simulink model "LQ_6DOF_V3"  (R2025b)
settings: Solver=VariableStepAuto  StartTime=0.0  StopTime=27.7  RelTol=1e-3
undefined symbols (not defined in the file): AVI, bp, cg, dcg_dMfu_table, dcg_dMox_table, dI_dMfu_table, dI_dMox_table, ENGINE, fu_masses, IN, K1flat, K2grid, MoI, OUT, ox_masses, TANKS, Target_Trajectory, tbl1, tbl2, tgrid, unom
libraries: aerolibanim x1, dspindex x1, matrix_library x1
settings Model: Creator=maxma  LastModifiedBy=maxma

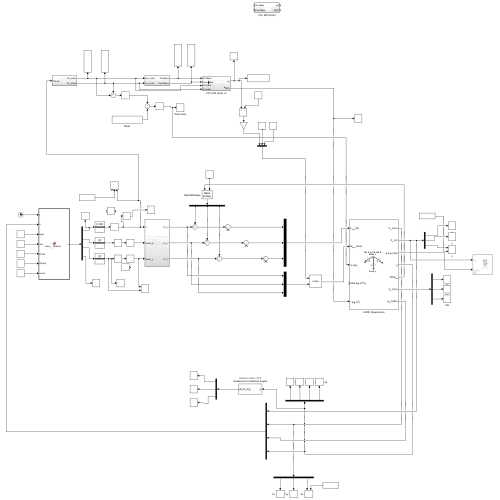
[thumbnail: Simulink's stored preview of the top-level diagram]
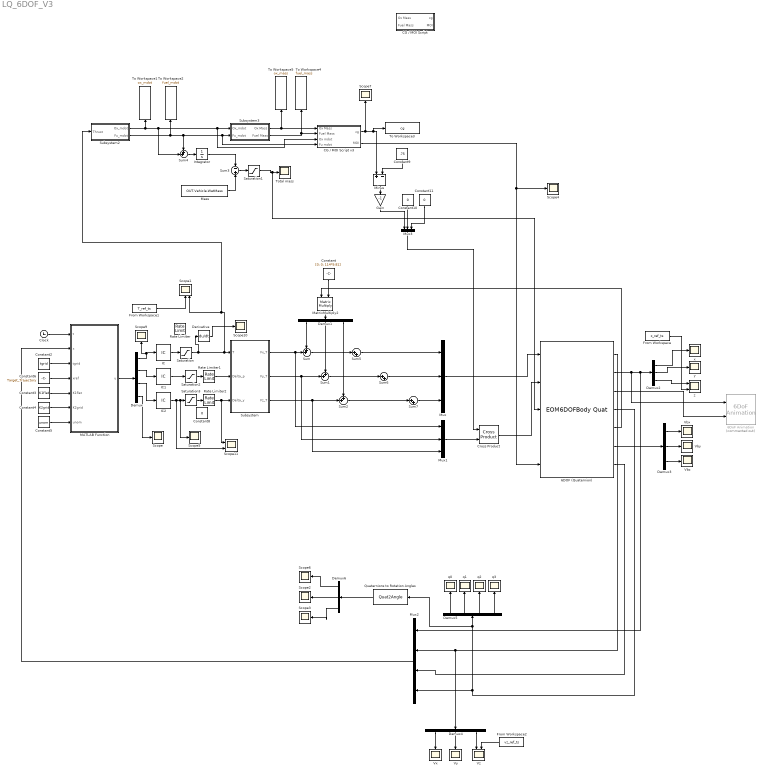
== system LQ_6DOF_V3 ==
  6DOF (Quaternion) : EOM6DOFBodyQuat  mtype=Custom Variable  eul_0=[pi/16 pi/2 pi/16]  mass_0=114  inertia=[16.5 0 0; 0 16.5 0; 0 0 16.5]
  6DoF Animation : aerolibanim/6DoF Animation  Commented=on  u1=[0 200 -200 200 -100 5]  u2=0.1  u3=2  u4=[4000 0 -5000]  u5=Fly alongside  u6=[100 100 -50]  u7=10  u8=on
  CG / MOI Script : Subsystem
  CG / MOI Script v3 : Subsystem
  Clock : Clock
  Constant : Constant  Value=[0; 0; 114*9.81]
  Constant10 : Constant  Value=0
  Constant11 : Constant  Value=0
  Constant2 : Constant  Value=tgrid
  Constant3 : Constant  Value=K1flat
  Constant4 : Constant  Value=K2grid
  Constant5 : Constant  Value=unom
  Constant6 : Constant  Value=Target_Trajectory
  Constant8 : Constant  Value=0
  Constant9 : Constant  Value=.75
  Cross Product : matrix_library/Cross Product
  Demux : Demux
  Demux{1..4,6} (5 alike) : Demux  Outputs=3
  Demux5 : Demux
  Derivative : Derivative  CoefficientInTFapproximation=10^-3
  From Workspace : FromWorkspace  VariableName=z_ref_ts
  From Workspace1 : FromWorkspace  VariableName=T_ref_ts
  From Workspace2 : FromWorkspace  VariableName=vz_ref_ts
  Gain : Gain  Gain=-1
  IC : InitialCondition  Value=1300
  IC1 : InitialCondition  Value=0
  IC2 : InitialCondition  Value=0
  Integrator : Integrator
  MATLAB Function : MATLAB Function  TreatAsAtomicUnit=on
  Mass : Constant  Value=OUT.Vehicle.WetMass
  MatrixMultiply2 : Product  Multiplication=Matrix(*)
  Minus : Sum  Inputs=+-
  Mux : Mux  Inputs=3
  Mux1 : Mux  Inputs=3
  Mux2 : Mux
  Mux3 : Mux  Inputs=3
  Quaternions to Rotation Angles : Quat2Angle
      settings: AttributesFormatString=Rotation Order: %<rotationOrder>
  Rate Limiter : RateLimiter  RisingSlewLimit=400  FallingSlewLimit=-400  SampleTimeMode=inherited
  Rate Limiter1 : RateLimiter  RisingSlewLimit=30*(pi/180)  FallingSlewLimit=-30*(pi/180)  SampleTimeMode=inherited
  Rate Limiter2 : RateLimiter  RisingSlewLimit=30*(pi/180)  FallingSlewLimit=-30*(pi/180)  SampleTimeMode=inherited
  Saturation : Saturate  UpperLimit=2400  LowerLimit=890
  Saturation1 : Saturate  UpperLimit=OUT.Vehicle.WetMass  LowerLimit=OUT.Vehicle.DryMass
  Saturation2 : Saturate  UpperLimit=7.5*(pi/180)  LowerLimit=-7.5*(pi/180)
  Saturation3 : Saturate  UpperLimit=7.5*(pi/180)  LowerLimit=-7.5*(pi/180)
  Scope{,2..7,9..10} (9 alike) : Scope
      Scope settings: ActiveDisplayYMinimum=-3.0324843779906377E-12  ActiveDisplayYMaximum=5.2601576594002828E-13  DataLoggingVariableName=ScopeData16
      Scope10 settings: ActiveDisplayYMinimum=-65.775875066860962  ActiveDisplayYMaximum=70.502667630153027  DataLoggingVariableName=ScopeData25
      Scope2 settings: ActiveDisplayYMinimum=1.5707657022295076  ActiveDisplayYMaximum=1.5707997295243843  DataLoggingVariableName=ScopeData17
      Scope3 settings: ActiveDisplayYMinimum=-3.9269859448764697  ActiveDisplayYMaximum=3.926989958417944  DataLoggingVariableName=ScopeData18
      Scope4 settings: ActiveDisplayYMinimum=-4.8001439667860453  ActiveDisplayYMaximum=43.201295701074415  DataLoggingVariableName=ScopeData4
      Scope5 settings: ActiveDisplayYMinimum=-1  ActiveDisplayYMaximum=1  DataLoggingVariableName=ScopeData5
      Scope6 settings: ActiveDisplayYMinimum=-3.9269859448764652  ActiveDisplayYMaximum=3.9269899584179448  DataLoggingVariableName=ScopeData19
      Scope7 settings: ActiveDisplayYMinimum=0.92832100501550818  ActiveDisplayYMaximum=1.0480775142034395  DataLoggingVariableName=ScopeData20
      Scope9 settings: DataLoggingVariableName=ScopeData24
  Scope1 : Scope  NumInputPorts=3
      settings: ActiveDisplayYMinimum=-771.02753736758768  ActiveDisplayYMaximum=3013.6766717670284
  Scope11 : Scope  NumInputPorts=2
      settings: ActiveDisplayYMinimum=-2.8831472481064673E-8  ActiveDisplayYMaximum=2.8689575203909038E-8  DataLoggingVariableName=ScopeData26
  Subsystem : Subsystem
  Subsystem2 : Subsystem
  Subsystem3 : Subsystem
  Sum{,1..2,4} (4 alike) : Sum  Inputs=++|
  Sum3 : Sum  Inputs=-|+
  Sum5 : Sum  Inputs=|++
  Sum6 : Sum  Inputs=|++
  Sum7 : Sum  Inputs=|++
  To Workspace1 : ToWorkspace  VariableName=ox_mdot  SaveFormat=Timeseries  SampleTime=-1
  To Workspace2 : ToWorkspace  VariableName=fuel_mdot  SaveFormat=Timeseries  SampleTime=-1
  To Workspace3 : ToWorkspace  VariableName=cg  SaveFormat=Timeseries  SampleTime=-1
  To Workspace4 : ToWorkspace  VariableName=fuel_mass  SaveFormat=Timeseries  SampleTime=-1
  To Workspace5 : ToWorkspace  VariableName=ox_mass  SaveFormat=Timeseries  SampleTime=-1
  Total mass : Scope
      settings: ActiveDisplayYMinimum=13.754311330723397  ActiveDisplayYMaximum=213.7543113307234  DataLoggingVariableName=ScopeData23
  Vbx : Scope
      settings: ActiveDisplayYMinimum=-1  ActiveDisplayYMaximum=1  DataLoggingVariableName=ScopeData6
  Vby : Scope
      settings: ActiveDisplayYMinimum=-1  ActiveDisplayYMaximum=1  DataLoggingVariableName=ScopeData7
  Vbz : Scope
      settings: ActiveDisplayYMinimum=-1  ActiveDisplayYMaximum=1  DataLoggingVariableName=ScopeData8
  Vx : Scope
      settings: ActiveDisplayYMinimum=-1  ActiveDisplayYMaximum=1  DataLoggingVariableName=ScopeData9
  Vy : Scope
      settings: DataLoggingVariableName=ScopeData10
  Vz : Scope  NumInputPorts=2
      settings: ActiveDisplayYMinimum=-7.8986716750089583  ActiveDisplayYMaximum=3.7459269640586941  DataLoggingVariableName=ScopeData11
  q{0..3} (4 alike) : Scope
      q0 settings: ActiveDisplayYMinimum=-1  ActiveDisplayYMaximum=1  DataLoggingVariableName=ScopeData12
      q1 settings: ActiveDisplayYMinimum=-1  ActiveDisplayYMaximum=1  DataLoggingVariableName=ScopeData13
      q2 settings: ActiveDisplayYMinimum=-1  ActiveDisplayYMaximum=1  DataLoggingVariableName=ScopeData14
      q3 settings: ActiveDisplayYMinimum=-1  ActiveDisplayYMaximum=1  DataLoggingVariableName=ScopeData15
  x : Scope
      settings: ActiveDisplayYMinimum=-1  ActiveDisplayYMaximum=1
  y : Scope
      settings: ActiveDisplayYMinimum=-1  ActiveDisplayYMaximum=1  DataLoggingVariableName=ScopeData2
  z : Scope  NumInputPorts=2
      settings: ActiveDisplayYMinimum=-33.672522393176216  ActiveDisplayYMaximum=3.7425921324673848  DataLoggingVariableName=ScopeData3
  wires:
  6DOF (Quaternion)/2 -> 6DoF Animation/1, Demux2/1, Mux2/1
  Subsystem/1(Fx_T) -> Sum/2, Mux1/1
  Subsystem/2(Fy_T) -> Sum1/2, Mux1/2
  Subsystem/3(Fz_T) -> Sum2/2, Mux1/3
  Mux/1 -> 6DOF (Quaternion)/1
  MatrixMultiply2/1 -> Demux1/1
  Cross Product/1 -> 6DOF (Quaternion)/2
  6DOF (Quaternion)/5 -> MatrixMultiply2/1
  6DOF (Quaternion)/6 -> Demux3/1
  6DOF (Quaternion)/7 -> Mux2/3
  6DOF (Quaternion)/1 -> Demux4/1, Mux2/2
  6DOF (Quaternion)/4 -> Mux2/4, Quaternions to Rotation Angles/1, Demux5/1
  MATLAB Function/1(u) -> Demux/1
  Demux/1 -> Scope9/1, IC/1
  Demux/2 -> IC1/1
  Demux/3 -> IC2/1
  Mux2/1 -> MATLAB Function/2(x)
  Constant2/1 -> MATLAB Function/3(tgrid)
  Clock/1 -> MATLAB Function/1(t)
  Constant6/1 -> MATLAB Function/4(xref)
  Constant3/1 -> MATLAB Function/5(K1flat)
  Constant4/1 -> MATLAB Function/6(K2grid)
  Constant5/1 -> MATLAB Function/7(unom)
  Constant/1 -> MatrixMultiply2/2
  IC2/1 -> Scope11/2, Scope5/1, Saturation3/1
  IC1/1 -> Saturation2/1
  IC/1 -> Saturation/1
  Demux1/1 -> Sum/1
  Demux1/2 -> Sum1/1
  Demux1/3 -> Sum2/1
  6DOF (Quaternion)/3 -> 6DoF Animation/2
  Demux2/1 -> x/1
  Demux2/2 -> y/1
  Demux2/3 -> z/1
  Demux3/3 -> Vbz/1
  Demux3/2 -> Vby/1
  Demux3/1 -> Vbx/1
  Demux4/1 -> Vx/1
  Demux4/2 -> Vy/1
  Demux4/3 -> Vz/1
  Demux5/2 -> q1/1
  Demux5/4 -> q3/1
  Demux5/3 -> q2/1
  Demux5/1 -> q0/1
  From Workspace/1 -> z/2
  From Workspace1/1 -> Scope1/2
  Demux/4 -> Scope/1
  Mux1/1 -> Cross Product/2
  From Workspace2/1 -> Vz/2
  Quaternions to Rotation Angles/1 -> Demux6/1
  Demux6/2 -> Scope2/1
  Demux6/3 -> Scope3/1
  Demux6/1 -> Scope6/1
  Sum3/1 -> Saturation1/1
  Subsystem3/2(Fuel Mass) -> CG / MOI Script v3/2(Fuel Mass), To Workspace4/1
  Saturation1/1 -> 6DOF (Quaternion)/3, Total mass/1
  Mass/1 -> Sum3/2
  Subsystem3/1(Ox Mass) -> CG / MOI Script v3/1(Ox Mass), To Workspace5/1
  Integrator/1 -> Sum3/1
  Subsystem2/1(Ox_mdot) -> To Workspace1/1, CG / MOI Script v3/3(Ox mdot), Subsystem3/1(Ox_mdot), Sum4/2
  Subsystem2/2(Fu_mdot) -> CG / MOI Script v3/4(Fu mdot), Subsystem3/2(Fu_mdot), Sum4/1, To Workspace2/1
  Sum4/1 -> Integrator/1
  Constant9/1 -> Minus/2
  Minus/1 -> Gain/1
  Gain/1 -> Mux3/1
  Constant10/1 -> Mux3/2
  Constant11/1 -> Mux3/3
  Mux3/1 -> Cross Product/1
  CG / MOI Script v3/1(cg) -> Minus/1, To Workspace3/1, Scope7/1
  CG / MOI Script v3/2(MOI) -> Scope4/1, 6DOF (Quaternion)/5
  Saturation2/1 -> Rate Limiter1/1
  Saturation3/1 -> Rate Limiter2/1
  Sum/1 -> Sum5/1
  Sum5/1 -> Mux/1
  Sum1/1 -> Sum6/1
  Sum6/1 -> Mux/2
  Sum7/1 -> Mux/3
  Sum2/1 -> Sum7/1
  Rate Limiter1/1 -> Subsystem/2(Delta_p)
  Rate Limiter2/1 -> Scope11/1, Subsystem/3(Delta_y)
  Derivative/1 -> Scope10/1
  Saturation/1 -> Subsystem/1(T), Subsystem2/1(Thrust), Scope1/3, Derivative/1

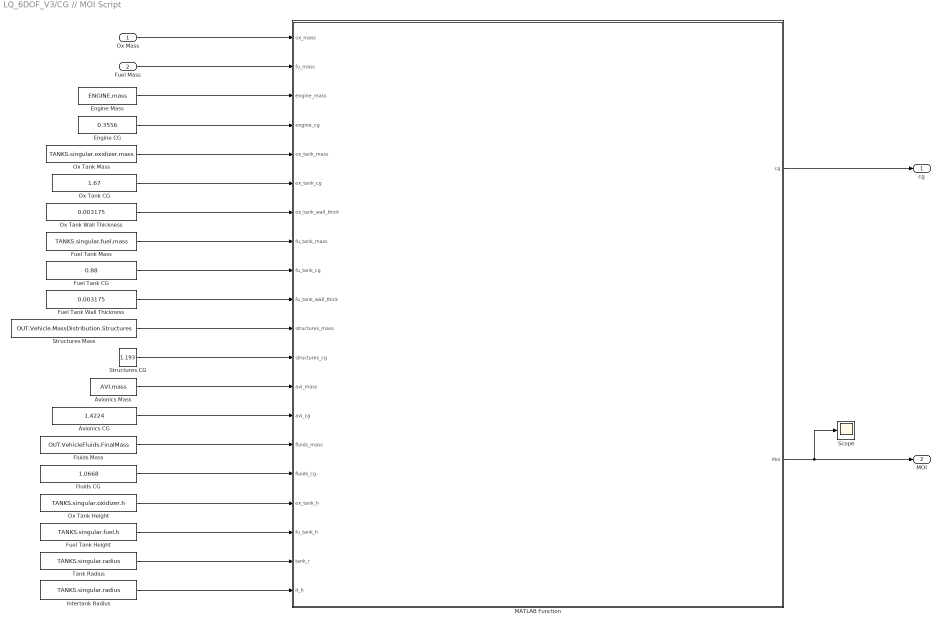
== system LQ_6DOF_V3/CG // MOI Script ==
  Ox Mass : Inport
  Fuel Mass : Inport  Port=2
  Avionics CG : Constant  Value=1.4224
  Avionics Mass : Constant  Value=AVI.mass
  Engine CG : Constant  Value=0.3556
  Engine Mass : Constant  Value=ENGINE.mass
  Fluids CG : Constant  Value=1.0668
  Fluids Mass : Constant  Value=OUT.VehicleFluids.FinalMass
  Fuel Tank CG : Constant  Value=0.88
  Fuel Tank Height : Constant  Value=TANKS.singular.fuel.h
  Fuel Tank Mass : Constant  Value=TANKS.singular.fuel.mass
  Fuel Tank Wall Thickness : Constant  Value=0.003175
  Intertank Radius : Constant  Value=TANKS.singular.radius
  MATLAB Function : MATLAB Function  TreatAsAtomicUnit=on
  Ox Tank CG : Constant  Value=1.67
  Ox Tank Height : Constant  Value=TANKS.singular.oxidizer.h
  Ox Tank Mass : Constant  Value=TANKS.singular.oxidizer.mass
  Ox Tank Wall Thickness : Constant  Value=0.003175
  Scope : Scope
      settings: DataLoggingVariableName=ScopeData16
  Structures CG : Constant  Value=1.193
  Structures Mass : Constant  Value=OUT.Vehicle.MassDistribution.Structures
  Tank Radius : Constant  Value=TANKS.singular.radius
  cg : Outport
  MOI : Outport  Port=2
  wires:
  Ox Mass/1 -> MATLAB Function/1(ox_mass)
  Fuel Mass/1 -> MATLAB Function/2(fu_mass)
  Engine Mass/1 -> MATLAB Function/3(engine_mass)
  Engine CG/1 -> MATLAB Function/4(engine_cg)
  Ox Tank Mass/1 -> MATLAB Function/5(ox_tank_mass)
  Ox Tank CG/1 -> MATLAB Function/6(ox_tank_cg)
  Ox Tank Wall Thickness/1 -> MATLAB Function/7(ox_tank_wall_thick)
  Fuel Tank Mass/1 -> MATLAB Function/8(fu_tank_mass)
  Fuel Tank CG/1 -> MATLAB Function/9(fu_tank_cg)
  Fuel Tank Wall Thickness/1 -> MATLAB Function/10(fu_tank_wall_thick)
  Structures Mass/1 -> MATLAB Function/11(structures_mass)
  Structures CG/1 -> MATLAB Function/12(structures_cg)
  Avionics Mass/1 -> MATLAB Function/13(avi_mass)
  Avionics CG/1 -> MATLAB Function/14(avi_cg)
  Fluids Mass/1 -> MATLAB Function/15(fluids_mass)
  Fluids CG/1 -> MATLAB Function/16(fluids_cg)
  Ox Tank Height/1 -> MATLAB Function/17(ox_tank_h)
  Fuel Tank Height/1 -> MATLAB Function/18(fu_tank_h)
  Tank Radius/1 -> MATLAB Function/19(tank_r)
  Intertank Radius/1 -> MATLAB Function/20(it_h)
  MATLAB Function/2(MoI) -> Scope/1, MOI/1
  MATLAB Function/1(cg) -> cg/1

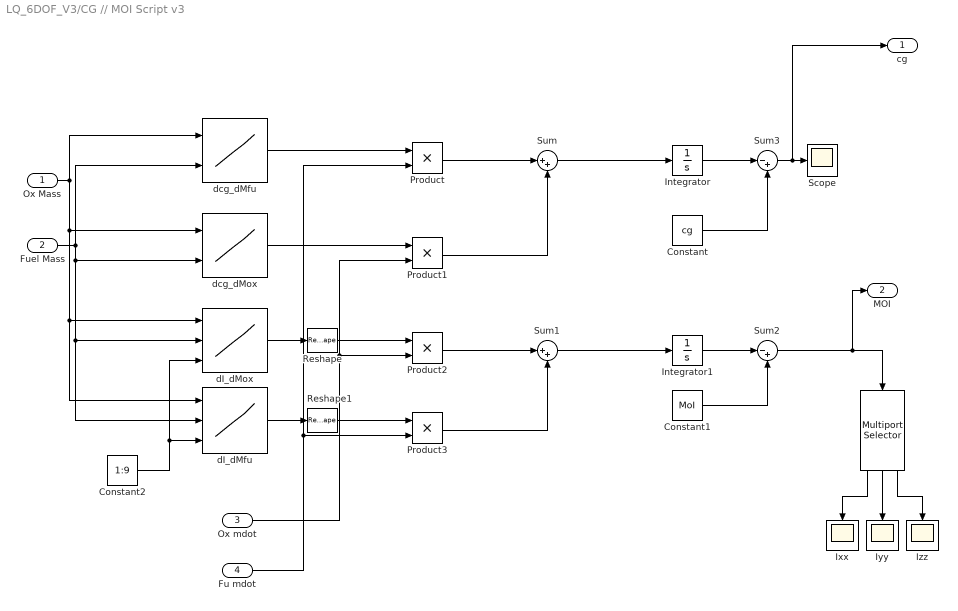
== system LQ_6DOF_V3/CG // MOI Script v3 ==
  Ox Mass : Inport
  Fuel Mass : Inport  Port=2
  Ox mdot : Inport  Port=3
  Fu mdot : Inport  Port=4
  " " : dspindex/Multiport Selector  rowsOrCols=Rows  idxCellArray={1,2,3}  idxErrMode=Clip Index
      settings: LibrarySourceBlock=|
      | dsphdlsupportsigmgmt/Multiport
      | Selector
  Constant : Constant  Value=cg
  Constant1 : Constant  Value=MoI
  Constant2 : Constant  Value=1:9
  Integrator : Integrator
  Integrator1 : Integrator
  Ixx : Scope
      settings: ActiveDisplayYMinimum=-0.12644047609192863  ActiveDisplayYMaximum=1.1379642848273579  DataLoggingVariableName=ScopeData19
  Iyy : Scope
      settings: ActiveDisplayYMinimum=30.163212884427733  ActiveDisplayYMaximum=49.780093450314517  DataLoggingVariableName=ScopeData20
  Izz : Scope
      settings: ActiveDisplayYMinimum=-2.8210574648941242  ActiveDisplayYMaximum=25.389517184047122  DataLoggingVariableName=ScopeData22
  Product{,1..3} (4 alike) : Product
  Reshape : Reshape  OutputDimensionality=Customize  OutputDimensions=[3,3]
  Reshape1 : Reshape  OutputDimensionality=Customize  OutputDimensions=[3,3]
  Scope : Scope
      settings: ActiveDisplayYMinimum=-1  ActiveDisplayYMaximum=1  DataLoggingVariableName=ScopeData18
  Sum : Sum  Inputs=|++
  Sum1 : Sum  Inputs=|++
  Sum2 : Sum  Inputs=|-+
  Sum3 : Sum  Inputs=|-+
  dI_dMfu : Lookup_n-D  NumberOfTableDimensions=3  BreakpointsForDimension1=ox_masses  BreakpointsForDimension2=fu_masses  BreakpointsForDimension3=1:9  Table=dI_dMfu_table  InternalRulePriority=Speed  RndMeth=Simplest
      settings: InputPortMap=u0,u1,u2
  dI_dMox : Lookup_n-D  NumberOfTableDimensions=3  BreakpointsForDimension1=ox_masses  BreakpointsForDimension2=fu_masses  BreakpointsForDimension3=1:9  Table=dI_dMox_table  InternalRulePriority=Speed  RndMeth=Simplest
      settings: InputPortMap=u0,u1,u2
  dcg_dMfu : Lookup_n-D  BreakpointsForDimension1=ox_masses  BreakpointsForDimension2=fu_masses  BreakpointsForDimension3=[5, 7]  Table=dcg_dMfu_table  InternalRulePriority=Speed  RndMeth=Simplest
      settings: InputPortMap=u0,u1
  dcg_dMox : Lookup_n-D  BreakpointsForDimension1=ox_masses  BreakpointsForDimension2=fu_masses  BreakpointsForDimension3=[5, 7]  Table=dcg_dMox_table  InternalRulePriority=Speed  RndMeth=Simplest
      settings: InputPortMap=u0,u1
  cg : Outport
  MOI : Outport  Port=2
  wires:
  Ox Mass/1 -> dI_dMfu/1, dI_dMox/1, dcg_dMox/1, dcg_dMfu/1
  Fuel Mass/1 -> dI_dMfu/2, dI_dMox/2, dcg_dMox/2, dcg_dMfu/2
  dcg_dMfu/1 -> Product/1
  Ox mdot/1 -> Product2/2, Product1/2
  dcg_dMox/1 -> Product1/1
  Fu mdot/1 -> Product3/2, Product/2
  dI_dMox/1 -> Reshape/1
  dI_dMfu/1 -> Reshape1/1
  Product/1 -> Sum/1
  Product1/1 -> Sum/2
  Product2/1 -> Sum1/1
  Product3/1 -> Sum1/2
  Sum/1 -> Integrator/1
  Integrator/1 -> Sum3/1
  Constant/1 -> Sum3/2
  Sum3/1 -> cg/1, Scope/1
  Sum1/1 -> Integrator1/1
  Integrator1/1 -> Sum2/1
  Constant1/1 -> Sum2/2
  Reshape/1 -> Product2/1
  Reshape1/1 -> Product3/1
  Constant2/1 -> dI_dMfu/3, dI_dMox/3
  " "/2 -> Iyy/1
  " "/1 -> Ixx/1
  " "/3 -> Izz/1
  Sum2/1 -> MOI/1, " "/1

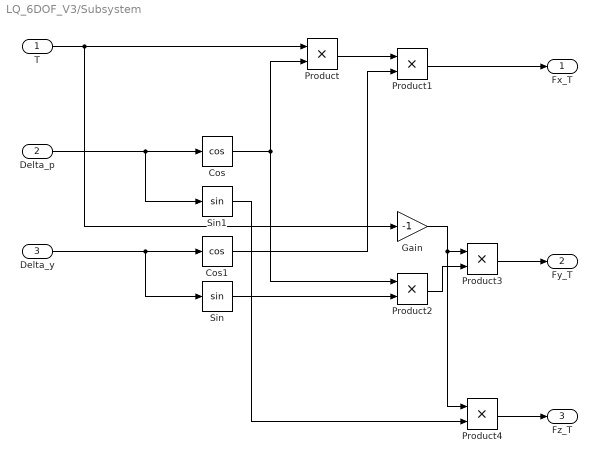
== system LQ_6DOF_V3/Subsystem ==
  T : Inport
  Delta_p : Inport  Port=2
  Delta_y : Inport  Port=3
  Cos : Trigonometry  Operator=cos
  Cos1 : Trigonometry  Operator=cos
  Gain : Gain  Gain=-1
  Product{,1..4} (5 alike) : Product
  Sin : Trigonometry
  Sin1 : Trigonometry
  Fx_T : Outport
  Fy_T : Outport  Port=2
  Fz_T : Outport  Port=3
  wires:
  Delta_p/1 -> Sin1/1, Cos/1
  T/1 -> Gain/1, Product/1
  Product/1 -> Product1/1
  Cos/1 -> Product2/1, Product/2
  Delta_y/1 -> Sin/1, Cos1/1
  Cos1/1 -> Product1/2
  Product1/1 -> Fx_T/1
  Sin/1 -> Product2/2
  Gain/1 -> Product4/1, Product3/1
  Product2/1 -> Product3/2
  Product3/1 -> Fy_T/1
  Sin1/1 -> Product4/2
  Product4/1 -> Fz_T/1

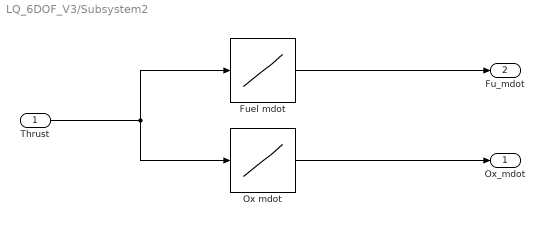
== system LQ_6DOF_V3/Subsystem2 ==
  Thrust : Inport
  Fuel mdot : Lookup_n-D  NumberOfTableDimensions=1  BreakpointsForDimension1=bp  Table=tbl2  InternalRulePriority=Speed  RndMeth=Simplest
  Ox mdot : Lookup_n-D  NumberOfTableDimensions=1  BreakpointsForDimension1=bp  Table=tbl1  InternalRulePriority=Speed  RndMeth=Simplest
  Ox_mdot : Outport
  Fu_mdot : Outport  Port=2
  wires:
  Thrust/1 -> Ox mdot/1, Fuel mdot/1
  Fuel mdot/1 -> Fu_mdot/1
  Ox mdot/1 -> Ox_mdot/1

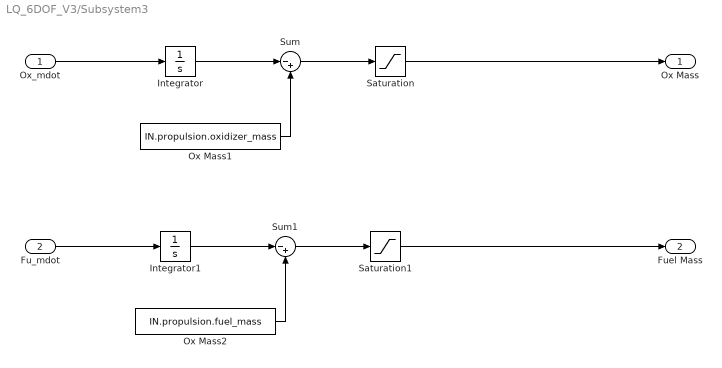
== system LQ_6DOF_V3/Subsystem3 ==
  Ox_mdot : Inport
  Fu_mdot : Inport  Port=2
  Integrator : Integrator
  Integrator1 : Integrator
  Ox Mass1 : Constant  Value=IN.propulsion.oxidizer_mass
  Ox Mass2 : Constant  Value=IN.propulsion.fuel_mass
  Saturation : Saturate  UpperLimit=IN.propulsion.oxidizer_mass  LowerLimit=0
  Saturation1 : Saturate  UpperLimit=IN.propulsion.fuel_mass  LowerLimit=0
  Sum : Sum  Inputs=|-+
  Sum1 : Sum  Inputs=|-+
  Ox Mass : Outport
  Fuel Mass : Outport  Port=2
  wires:
  Ox_mdot/1 -> Integrator/1
  Integrator/1 -> Sum/1
  Ox Mass1/1 -> Sum/2
  Sum/1 -> Saturation/1
  Saturation/1 -> Ox Mass/1
  Sum1/1 -> Saturation1/1
  Saturation1/1 -> Fuel Mass/1
  Fu_mdot/1 -> Integrator1/1
  Ox Mass2/1 -> Sum1/2
  Integrator1/1 -> Sum1/1

== matlab function LQ_6DOF_V3/CG // MOI Script/MATLAB Function ==
  data: ox_mass input; cg output; fu_mass input; engine_mass input; engine_cg input; ox_tank_mass input; ox_tank_cg input; ox_tank_wall_thick input; fu_tank_mass input; fu_tank_cg input; fu_tank_wall_thick input; structures_mass input; structures_cg input; avi_mass input; avi_cg input; fluids_mass input; fluids_cg input; ox_tank_h input; fu_tank_h input; tank_r input; it_h input; MoI output
function [cg, MoI] = cg_sim(ox_mass, fu_mass, engine_mass, engine_cg, ox_tank_mass, ox_tank_cg, ox_tank_wall_thick, fu_tank_mass, fu_tank_cg, fu_tank_wall_thick, structures_mass, structures_cg, avi_mass, avi_cg, fluids_mass, fluids_cg, ox_tank_h, fu_tank_h, tank_r, it_h)
%CG_SIM Calculates the Center of Gravity and Moment of Inertia Matrix
%   Inputs are masses (kg), CG positions (m), and dimensions (m).

    %% 1. Constants and Unit Conversions
        ox_density = 1141;   % kg/m^3
        fu_density = 800;    % kg/m^3
    al_density = 2700;   % kg/m^3 (Density of Al6061)
    
    % Engine dimensions: 4 inch radius, 1 ft length
    eng_r = 4 * 0.0254;  % inches to meters
    eng_h = 1 * 0.3048;  % ft to meters

    %% 2. End Cap Geometry & Mass (NEW)
    % Modeled as solid cylinders attached to the ends of the tank shells.
    % Height of cap = wall thickness of the respective tank.
    
    % --- Oxidizer Tank Caps ---
    h_ox_cap = ox_tank_wall_thick;
    vol_ox_cap = pi * tank_r^2 * h_ox_cap;
    m_ox_cap   = al_density * vol_ox_cap; % Mass of ONE cap
    
    % Positions (Top and Bottom of the hollow shell)
    % Z = Tank_CG +/- (Tank_H/2 + Cap_H/2)
    z_ox_cap_bot = ox_tank_cg - (ox_tank_h / 2) - (h_ox_cap / 2);
    z_ox_cap_top = ox_tank_cg + (ox_tank_h / 2) + (h_ox_cap / 2);

    % --- Fuel Tank Caps ---
    h_fu_cap = fu_tank_wall_thick;
    vol_fu_cap = pi * tank_r^2 * h_fu_cap;
    m_fu_cap   = al_density * vol_fu_cap; % Mass of ONE cap
    
    % Positions
    z_fu_cap_bot = fu_tank_cg - (fu_tank_h / 2) - (h_fu_cap / 2);
    z_fu_cap_top = fu_tank_cg + (fu_tank_h / 2) + (h_fu_cap / 2);

    %% 3. Fluid Geometry Calculations
    % Fuel Fluid
    if fu_mass > 0
        h_fu_fluid = (fu_mass / fu_density) / (pi * tank_r^2);
        % Fluid sits at the bottom of the tank shell
        z_fu_fluid = (fu_tank_cg - fu_tank_h/2) + (h_fu_fluid / 2);
    else
        h_fu_fluid = 0; z_fu_fluid = 0;
    end

    % Oxidizer Fluid
    if ox_mass > 0
        h_ox_fluid = (ox_mass / ox_density) / (pi * tank_r^2);
        z_ox_fluid = (ox_tank_cg - ox_tank_h/2) + (h_ox_fluid / 2);
    else
        h_ox_fluid = 0; z_ox_fluid = 0;
    end

    %% 4. Calculate System Center of Gravity (CG)
    % Sum of Moments = sum(mass * position)
    moment_sum = ...
        engine_mass * engine_cg + ...
        fu_tank_mass * fu_tank_cg + ...
        ox_tank_mass * ox_tank_cg + ...
        structures_mass * structures_cg + ...
        avi_mass * avi_cg + ...
        fu_mass * z_fu_fluid + ...
        ox_mass * z_ox_fluid + ...
        m_ox_cap * z_ox_cap_bot + ... 
        m_ox_cap * z_ox_cap_top + ...  
        m_fu_cap * z_fu_cap_bot + ...  
        m_fu_cap * z_fu_cap_top;      

    total_mass = engine_mass + fu_tank_mass + ox_tank_mass + ...
                 structures_mass + avi_mass + fu_mass + ox_mass + ...
                 2 * m_ox_cap + 2 * m_fu_cap;

    if total_mass > 0
        cg = moment_sum / total_mass; % return 1
    else
        cg = 0;
    end

    %% 5. Calculate Moments of Inertia (MoI)
    % Anonymous functions for inertia - shout out gemini for this one
    calc_solid_Izz = @(m, r) 0.5 * m * r^2;
    calc_solid_Ixx = @(m, r, h) (1/12) * m * (3*r^2 + h^2);
    calc_hollow_Izz = @(m, ro, ri) 0.5 * m * (ro^2 + ri^2);
    calc_hollow_Ixx = @(m, ro, ri, h) (1/12) * m * (3*(ro^2 + ri^2) + h^2);

    % --- A. Engine ---
    Izz_eng = calc_solid_Izz(engine_mass, eng_r);
    Ixx_eng = calc_solid_Ixx(engine_mass, eng_r, eng_h) + engine_mass * (engine_cg - cg)^2;

    % --- B. Fuel Tank (Hollow Shell) ---
    r_in_fu = tank_r - fu_tank_wall_thick;
    Izz_fut = calc_hollow_Izz(fu_tank_mass, tank_r, r_in_fu);
    Ixx_fut = calc_hollow_Ixx(fu_tank_mass, tank_r, r_in_fu, fu_tank_h) + fu_tank_mass * (fu_tank_cg - cg)^2;

    % --- C. Oxidizer Tank (Hollow Shell) ---
    r_in_ox = tank_r - ox_tank_wall_thick;
    Izz_oxt = calc_hollow_Izz(ox_tank_mass, tank_r, r_in_ox);
    Ixx_oxt = calc_hollow_Ixx(ox_tank_mass, tank_r, r_in_ox, ox_tank_h) + ox_tank_mass * (ox_tank_cg - cg)^2;

    % --- D. Structures --- just asssume cylinder in it
    Izz_str = calc_solid_Izz(structures_mass, tank_r);
    Ixx_str = calc_solid_Ixx(structures_mass, tank_r, it_h) + structures_mass * (structures_cg - cg)^2;

    % --- E. Avionics --- just asssume cylinder in it
    Izz_avi = calc_solid_Izz(avi_mass, tank_r);
    Ixx_avi = calc_solid_Ixx(avi_mass, tank_r, it_h) + avi_mass * (avi_cg - cg)^2;

    % --- F. Fluids ---
    if fu_mass > 0
        Izz_fuf = calc_solid_Izz(fu_mass, tank_r);
        Ixx_fuf = calc_solid_Ixx(fu_mass, tank_r, h_fu_fluid) + fu_mass * (z_fu_fluid - cg)^2;
    else
        Izz_fuf = 0; Ixx_fuf = 0;
    end

    if ox_mass > 0
        Izz_oxf = calc_solid_Izz(ox_mass, tank_r);
        Ixx_oxf = calc_solid_Ixx(ox_mass, tank_r, h_ox_fluid) + ox_mass * (z_ox_fluid - cg)^2;
    else
        Izz_oxf = 0; Ixx_oxf = 0;
    end

    % --- G. End Caps ---
    % 1. Ox Caps (Solid Cylinders)
    % Izz is same for both
    Izz_ox_cap = calc_solid_Izz(m_ox_cap, tank_r);
    Ixx_ox_cap_local = calc_solid_Ixx(m_ox_cap, tank_r, h_ox_cap);
    
    Ixx_ox_caps_total = ...
        (Ixx_ox_cap_local + m_ox_cap * (z_ox_cap_bot - cg)^2) + ... % Bottom Cap
        (Ixx_ox_cap_local + m_ox_cap * (z_ox_cap_top - cg)^2);      % Top Cap

    % 2. Fuel Caps (Solid Cylinders)
    Izz_fu_cap = calc_solid_Izz(m_fu_cap, tank_r);
    Ixx_fu_cap_local = calc_solid_Ixx(m_fu_cap, tank_r, h_fu_cap);
    
    Ixx_fu_caps_total = ...
        (Ixx_fu_cap_local + m_fu_cap * (z_fu_cap_bot - cg)^2) + ... % Bottom Cap
        (Ixx_fu_cap_local + m_fu_cap * (z_fu_cap_top - cg)^2);      % Top Cap

    %% 6. Summation
    Izz_total = Izz_eng + Izz_fut + Izz_oxt + Izz_str + Izz_avi + ...
                Izz_fuf + Izz_oxf + ...
                2*Izz_ox_cap + 2*Izz_fu_cap;
                
    Ixx_total = Ixx_eng + Ixx_fut + Ixx_oxt + Ixx_str + Ixx_avi + ...
                Ixx_fuf + Ixx_oxf + ...
                Ixx_ox_caps_total + Ixx_fu_caps_total;
    
    Iyy_total = Ixx_total; % Symmetry

    MoI = [Izz_total, 0, 0; 
           0, Iyy_total, 0; 
           0, 0, Ixx_total]; % return 2
end

== matlab function LQ_6DOF_V3/MATLAB Function ==
  data: t input; u output; x input; tgrid input; xref input; K1flat input; K2grid input; unom input
function u = Gain_Selector(t, x, tgrid, xref, K1flat, K2grid, unom)
%#codegen
% Fixed-size output: u is always 4x1

u = zeros(4,1);

x = x(:);              % should be 13x1 for 6DOF
N = length(tgrid);

% --- Clamp time and compute interval index ---
if t <= tgrid(1)
    idx = 1;
    w = 0.0;
elseif t >= tgrid(end)
    idx = N-1;
    w = 1.0;
else
    idx = 1;
    for k = 1:(N-1)
        if tgrid(k) <= t && t < tgrid(k+1)
            idx = k;
            break;
        end
    end
    t1 = tgrid(idx);
    t2 = tgrid(idx+1);
    w  = (t - t1) / (t2 - t1);
end

% --- Interpolate reference state (13x1) ---
xref_t = (1-w)*xref(idx,:)' + w*xref(idx+1,:)';

% --- Interpolate K1flat then reshape to 4x13 ---
Kflat = (1-w)*K1flat(idx,:) + w*K1flat(idx+1,:);
K1 = reshape(Kflat, 13, 4)';   % 4x13   (requires K1flat is N×52)

% --- Interpolate K2 (4x1) ---
K2 = (1-w)*K2grid(idx,:)' + w*K2grid(idx+1,:)';

% --- Interpolate nominal control (4x1) ---
u_nom = (1-w)*unom(idx,:)' + w*unom(idx+1,:)';

% --- Control law ---
dx = (x - xref_t);          % 13x1
u  = u_nom - K1*dx - K2;    % try +K2 if thrust is mirrored

end
